simulink model "close_pid_dc_motor_v1_yedek"  (R2026a)
settings: Solver=VariableStepAuto  StopTime=25  MaxStep=0.01
InitFcn:
  | init_motor;
undefined symbols (not defined in the file or in its folder): motor
libraries: slpidlib x1
settings Model: Creator=seman  LastModifiedBy=seman

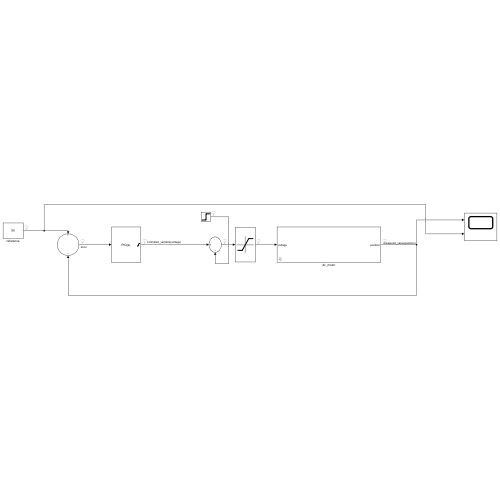
[thumbnail: Simulink's stored preview of the top-level diagram]
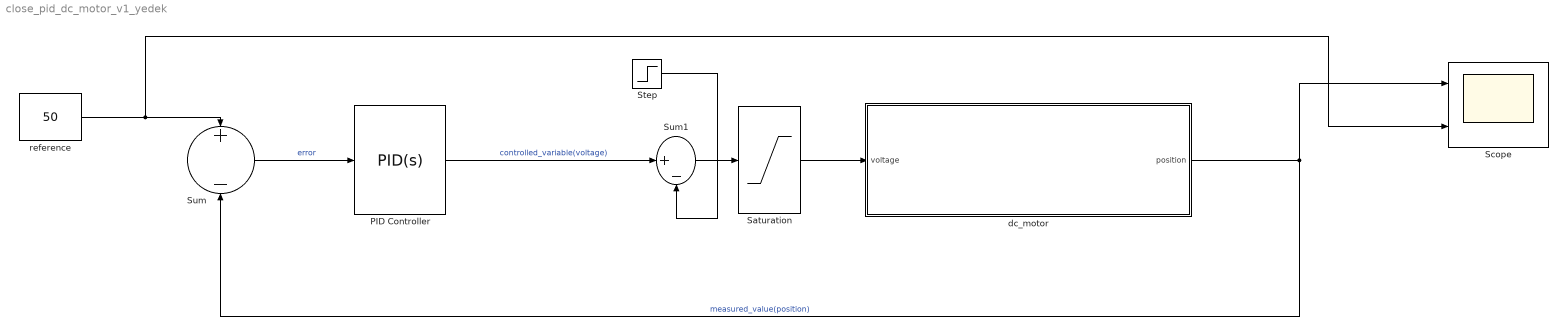
== system close_pid_dc_motor_v1_yedek ==
  PID Controller : slpidlib/PID Controller  Controller=PID  Form=Parallel  TimeDomain=Continuous-time  UseExternalTs=off  SampleTime=-1  IntegratorMethod=Forward Euler  FilterMethod=Forward Euler  ControllerParametersSource=internal  P=11.2299151129167  I=7.23044369863269  UseKiTs=off  D=4.16930526092153  UseExternalDerivativeSource=off  N=1010.41686394242  UseFilter=on  TunerSelectOption=Transfer Function Based (PID Tuner App)  InitialConditionSource=internal  InitialConditionForIntegrator=0  InitialConditionForFilter=0  DifferentiatorICPrevScaledInput=0  ExternalReset=none  TrackingMode=off  Kt=1  LimitOutput=on  SatLimitsSource=internal  UpperSaturationLimit=12  LowerSaturationLimit=-12  LinearizeAsGain=on  AntiWindupMode=back-calculation  Kb=1  LimitIntegrator=off  UpperIntegratorSaturationLimit=inf  LowerIntegratorSaturationLimit=-inf  POutMin=[]  POutMax=[]  IOutMin=[]  IOutMax=[]  DOutMin=[]  DOutMax=[]  NOutMin=[]  NOutMax=[]  SumOutMin=[]  SumOutMax=[]  SaturationOutMin=[]  SaturationOutMax=[]  PParamMin=[]  PParamMax=[]  IParamMin=[]  IParamMax=[]  DParamMin=[]  DParamMax=[]  NParamMin=[]  NParamMax=[]  KbParamMin=[]  KbParamMax=[]  KtParamMin=[]  KtParamMax=[]  KbOutMin=[]  KbOutMax=[]  KtOutMin=[]  KtOutMax=[]  IntegratorOutMin=[]  IntegratorOutMax=[]  FilterOutMin=[]  FilterOutMax=[]  SumI1OutMin=[]  SumI1OutMax=[]  SumI2OutMin=[]  SumI2OutMax=[]  SumI3OutMin=[]  SumI3OutMax=[]  SumI4OutMin=[]  SumI4OutMax=[]  SumDOutMin=[]  SumDOutMax=[]  DifferentiatorOutMin=[]  DifferentiatorOutMax=[]  FilterDiffOutCoefMin=[]  FilterDiffOutCoefMax=[]  ReciprocalOutMin=[]  ReciprocalOutMax=[]  SumDenOutMin=[]  SumDenOutMax=[]  SumNumOutMin=[]  SumNumOutMax=[]  DivideOutMin=[]  DivideOutMax=[]  UdiffTsProdOutMin=[]  UdiffTsProdOutMax=[]  NTsProdOutMin=[]  NTsProdOutMax=[]  UintegralTsProdOutMin=[]  UintegralTsProdOutMax=[]  UngainTsProdOutMin=[]  UngainTsProdOutMax=[]  ClampingZeroOutDataTypeStr=Inherit: Inherit via back propagation  ClampingZeroOutMin=[]  ClampingZeroOutMax=[]  FilterDenConstantOutDataTypeStr=Inherit: Inherit via back propagation  FilterDenConstantOutMin=[]  FilterDenConstantOutMax=[]  PCopyOutDataTypeStr=Inherit: Inherit via back propagation  PCopyOutMin=[]  PCopyOutMax=[]  NCopyOutDataTypeStr=Inherit: Inherit via back propagation  NCopyOutMin=[]  NCopyOutMax=[]  IntegratorContinuousStateAttributes=''  IntegratorStateMustResolveToSignalObject=off  IntegratorRTWStateStorageClass=Auto  FilterContinuousStateAttributes=''  FilterStateMustResolveToSignalObject=off  FilterRTWStateStorageClass=Auto  ParallelPVariant=InternalParameters  IdealPVariant=Disabled  IVariant=InternalParameters  DVariant=InternalParameters  IntegratorVariant=Continuous  SatVariant=Enabled  AWVariant=BackCalculation  PCopyVariant=Disabled  TRVariant=Disabled  FdbkBlocksVariant=Forward  IdealPFdbkVariant=Disabled  SatFdbkVariant=Disabled  DerivativeFilterVariant=ContFilter  NVariant=InternalParameters  NCopyVariant=Disabled  FilterICVariant=InternalICsFilter  IntegratorICVariant=InternalICs  ExternalResetVariant=Disabled  TRSumVariant=Passthrough  SumFdbkVariant=Disabled  SumVariant=Sum_PID  TsampFilterVariant=InternalTs  TsampNgainVariant=Passthrough  TsampIntegralVariant=Disabled_SignalSpec  ExternalSaturationOutDataTypeStr=Inherit: Same as second input  DerivativeSourceVariant=ErrorSignal  PreIntVariant=InternalPreInt
  Saturation : Saturate  UpperLimit=12  LowerLimit=-12
  Scope : Scope  NumInputPorts=2
      settings: ActiveDisplayYMinimum=-11.339350762490124  ActiveDisplayYMaximum=102.05415686241113
  Step : Step  Time=10  FinalValue=0  SampleTime=0
  Sum : Sum  Inputs=+-
  Sum1 : Sum  Inputs=|+-
  dc_motor : Subsystem  InitFcn=""  mask{J=1.2*motor.J, B=motor.B, KT=motor.KT, R=1.2*motor.R, L=motor.L, KB=motor.KB}
      mask prompts: J "J(KG*M^2)"; B "B(Nm/rad)"; KT "NM/AMPER"; R "R(OHM)"; L "L(H)"; KB "KB(VS/rad)"
  reference : Constant  Value=50
  wires:
  dc_motor/1(position) -> Scope/1, Sum/2  "measured_value(position)"
  reference/1 -> Scope/2, Sum/1
  Sum/1 -> PID Controller/1  "error"
  PID Controller/1 -> Sum1/1  "controlled_variable(voltage)"
  Saturation/1 -> dc_motor/1(voltage)
  Step/1 -> Sum1/2
  Sum1/1 -> Saturation/1

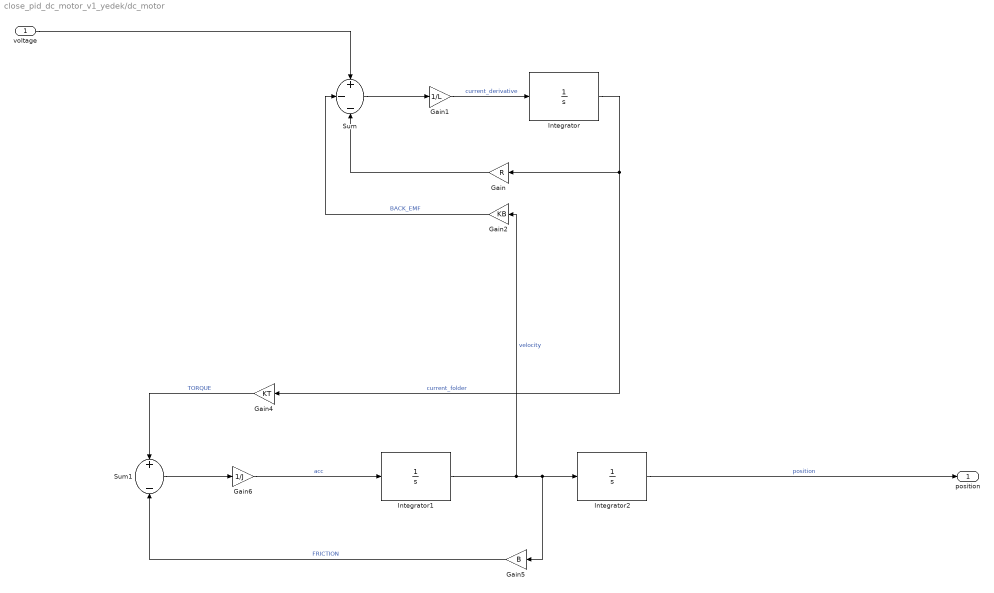
== system close_pid_dc_motor_v1_yedek/dc_motor ==
  voltage : Inport
  Gain : Gain  Gain=R
  Gain1 : Gain  Gain=1/L
  Gain2 : Gain  Gain=KB
  Gain4 : Gain  Gain=KT
  Gain5 : Gain  Gain=B
  Gain6 : Gain  Gain=1/J
  Integrator : Integrator
  Integrator1 : Integrator
  Integrator2 : Integrator
  Sum : Sum  Inputs=+--
  Sum1 : Sum  Inputs=+-
  position : Outport
  wires:
  Gain6/1 -> Integrator1/1  "acc"
  Integrator1/1 -> Gain2/1, Integrator2/1, Gain5/1  "velocity"
  Gain2/1 -> Sum/2  "BACK_EMF"
  Gain4/1 -> Sum1/1  "TORQUE"
  Integrator/1 -> Gain4/1, Gain/1  "current_folder"
  Gain/1 -> Sum/3
  Sum/1 -> Gain1/1
  Gain1/1 -> Integrator/1  "current_derivative"
  Sum1/1 -> Gain6/1
  Gain5/1 -> Sum1/2  "FRICTION"
  Integrator2/1 -> position/1  "position"
  voltage/1 -> Sum/1
